simulink model "solar_collector"  (R2025b)
settings: Solver=ode15s  StartTime=0  StopTime=LP.duration  MaxStep=5  RelTol=1e-7  AbsTol=1e-7
values from neighbouring files (symbols this model uses):
  P = g.P    [simulate_collector.m]
undefined symbols (not defined in the file or in its folder): LP
settings Model: Creator=aevamac  LastModifiedBy=aevamac
settings DataIOCC: SaveFormat=Array  OutputOption=SpecifiedOutputTimes  OutputTimes=LP.out_times

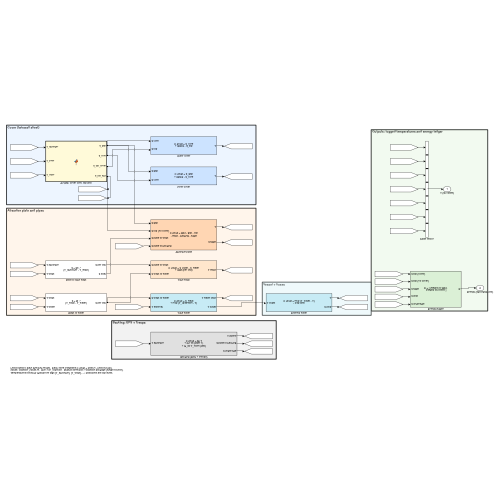
[thumbnail: Simulink's stored preview of the top-level diagram]
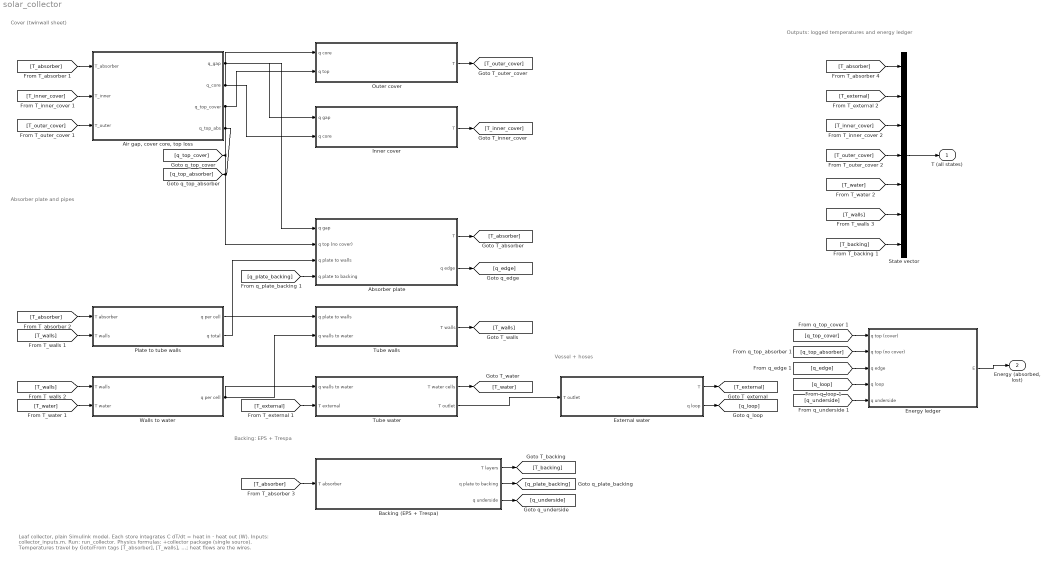
== system solar_collector ==
  note: Cover (twinwall sheet)
  note: Absorber plate and pipes
  note: Vessel + hoses
  note: Backing: EPS + Trespa
  note: Outputs: logged temperatures and energy ledger
  note: Leaf collector, plain Simulink model.  Each store integrates C dT/dt = heat in - heat out (W).
      | Inputs: collector_inputs.m.  Run: run_collector.  Physics formulas: +collector package (single source).
      | Temperatures travel by Goto/From tags [T_absorber], [T_walls], ...; heat flows are the wires.
  Absorber plate : Subsystem  Description=Aluminium plate + paint + tee fittings, one temperature. C dT/dt = (q_solar - q_tube) - q_gap - q_top(no cover) - sum q_plate->walls - q_plate->backing - edge loss
      mask Display:
      | disp(sprintf('C dT/dt = light - gap - top\n- walls - backing - edge'));
      | port_label('input', 1, 'q gap');
      | port_label('input', 2, 'q top (no cover)');
      | port_label('input', 3, 'q plate to walls');
      | port_label('input', 4, 'q plate to backing');
      | port_label('output', 1, 'T');
      | port_label('output', 2, 'q edge');
  "Air gap, cover core, top loss" : MATLAB Function  Description=Nonlinear surface heat flows from collector.surface_heat_flows: gap convection (Hollands-type correlation) + radiation, twinwall core conduction, and top loss by convection + radiation.  TreatAsAtomicUnit=on
  Backing (EPS + Trespa) : Subsystem  Description=EPS then the cart Trespa plate, each split into layers that store heat. Conduction plate -> layer 1 -> ... -> last layer -> underside air. Heat into the layers = Ab*Tb + G1*Ta (first) + G_air*T_room (last).
      mask Display:
      | disp(sprintf('C dT/dt = Ab T\n+ G1 Ta (layer 1)\n+ G_air T_room (last)'));
      | port_label('input', 1, 'T absorber');
      | port_label('output', 1, 'T layers');
      | port_label('output', 2, 'q plate to backing');
      | port_label('output', 3, 'q underside');
  Energy ledger : Subsystem  Description=Energy absorbed (light) and lost (top, edges, loop, underside), integrated so that absorbed - lost - stored can be checked (should be ~0).
      mask Display:
      | disp(sprintf('E = [ integral of light,\n integral of losses ]'));
      | port_label('input', 1, 'q top (cover)');
      | port_label('input', 2, 'q top (no cover)');
      | port_label('input', 3, 'q edge');
      | port_label('input', 4, 'q loop');
      | port_label('input', 5, 'q underside');
      | port_label('output', 1, 'E');
  External water : Subsystem  Description=Vessel and hoses, one mixed temperature. C dT/dt = mcp (T_outlet - Te) - loop_ua (Te - T_room)
      mask Display:
      | disp(sprintf('C dT/dt = mcp (T_outlet - T)\n- loop loss'));
      | port_label('input', 1, 'T outlet');
      | port_label('output', 1, 'T');
      | port_label('output', 2, 'q loop');
  Inner cover : Subsystem  Description=Inner cover sheet: C dT/dt = q_gap + q_cover/2 - q_core
      mask Display:
      | disp(sprintf('C dT/dt = q_gap\n+ light/2 - q_core'));
      | port_label('input', 1, 'q gap');
      | port_label('input', 2, 'q core');
      | port_label('output', 1, 'T');
  Outer cover : Subsystem  Description=Outer cover sheet: C dT/dt = q_core + q_cover/2 - q_top
      mask Display:
      | disp(sprintf('C dT/dt = q_core\n+ light/2 - q_top'));
      | port_label('input', 1, 'q core');
      | port_label('input', 2, 'q top');
      | port_label('output', 1, 'T');
  Plate to tube walls : Subsystem  Description=q = ga .* (T_absorber - T_walls), per cell; also the total leaving the plate
      mask Display:
      | disp(sprintf('q = ga .*\n(T_absorber - T_walls)'));
      | port_label('input', 1, 'T absorber');
      | port_label('input', 2, 'T walls');
      | port_label('output', 1, 'q per cell');
      | port_label('output', 2, 'q total');
  State vector : Concatenate  NumInputs=7
  Tube walls : Subsystem  Description=One LDPE wall cell per water cell. C dT/dt = ga(Ta - Tw) - gf(Tw - Tq) + light landing on the pipes (footprint share)
      mask Display:
      | disp(sprintf('C dT/dt = q_plate - q_water\n+ light (per cell)'));
      | port_label('input', 1, 'q plate to walls');
      | port_label('input', 2, 'q walls to water');
      | port_label('output', 1, 'T walls');
  Tube water : Subsystem  Description=Water cells in flow order (supply tiers, then the mirrored return). C dT/dt = gf(Tw - Tq) + mcp (T_upstream - Tq); the first cell is fed from the external water.
      mask Display:
      | disp(sprintf('C dT/dt = q_walls\n+ mcp (T_upstream - T)'));
      | port_label('input', 1, 'q walls to water');
      | port_label('input', 2, 'T external');
      | port_label('output', 1, 'T water cells');
      | port_label('output', 2, 'T outlet');
  Walls to water : Subsystem  Description=q = gf .* (T_walls - T_water), per cell
      mask Display:
      | disp(sprintf('q = gf .*\n(T_walls - T_water)'));
      | port_label('input', 1, 'T walls');
      | port_label('input', 2, 'T water');
      | port_label('output', 1, 'q per cell');
  T (all states) : Outport
  "Energy (absorbed, lost)" : Outport  Port=2
  wires:
  [T_absorber] -> "Air gap, cover core, top loss"/1(T_absorber)
  [T_inner_cover] -> "Air gap, cover core, top loss"/2(T_inner)
  [T_outer_cover] -> "Air gap, cover core, top loss"/3(T_outer)
  "Air gap, cover core, top loss"/1(q_gap) -> Inner cover/1(q gap), Absorber plate/1(q gap)
  "Air gap, cover core, top loss"/2(q_core) -> Inner cover/2(q core), Outer cover/1(q core)
  "Air gap, cover core, top loss"/3(q_top_cover) -> Outer cover/2(q top), [q_top_cover]
  Outer cover/1(T) -> [T_outer_cover]
  Inner cover/1(T) -> [T_inner_cover]
  "Air gap, cover core, top loss"/4(q_top_abs) -> [q_top_absorber], Absorber plate/2(q top (no cover))
  Absorber plate/1(T) -> [T_absorber]
  Absorber plate/2(q edge) -> [q_edge]
  [q_plate_backing] -> Absorber plate/4(q plate to backing)
  [T_absorber] -> Plate to tube walls/1(T absorber)
  [T_walls] -> Plate to tube walls/2(T walls)
  Plate to tube walls/1(q per cell) -> Tube walls/1(q plate to walls)
  Plate to tube walls/2(q total) -> Absorber plate/3(q plate to walls)
  Tube walls/1(T walls) -> [T_walls]
  [T_walls] -> Walls to water/1(T walls)
  [T_water] -> Walls to water/2(T water)
  Walls to water/1(q per cell) -> Tube walls/2(q walls to water), Tube water/1(q walls to water)
  [T_external] -> Tube water/2(T external)
  Tube water/1(T water cells) -> [T_water]
  Tube water/2(T outlet) -> External water/1(T outlet)
  External water/1(T) -> [T_external]
  External water/2(q loop) -> [q_loop]
  [T_absorber] -> Backing (EPS + Trespa)/1(T absorber)
  Backing (EPS + Trespa)/1(T layers) -> [T_backing]
  Backing (EPS + Trespa)/2(q plate to backing) -> [q_plate_backing]
  Backing (EPS + Trespa)/3(q underside) -> [q_underside]
  [q_top_cover] -> Energy ledger/1(q top (cover))
  [q_top_absorber] -> Energy ledger/2(q top (no cover))
  [q_edge] -> Energy ledger/3(q edge)
  [q_loop] -> Energy ledger/4(q loop)
  [q_underside] -> Energy ledger/5(q underside)
  Energy ledger/1(E) -> "Energy (absorbed, lost)"/1
  [T_absorber] -> State vector/1
  [T_external] -> State vector/2
  [T_inner_cover] -> State vector/3
  [T_outer_cover] -> State vector/4
  [T_water] -> State vector/5
  [T_walls] -> State vector/6
  [T_backing] -> State vector/7
  State vector/1 -> T (all states)/1

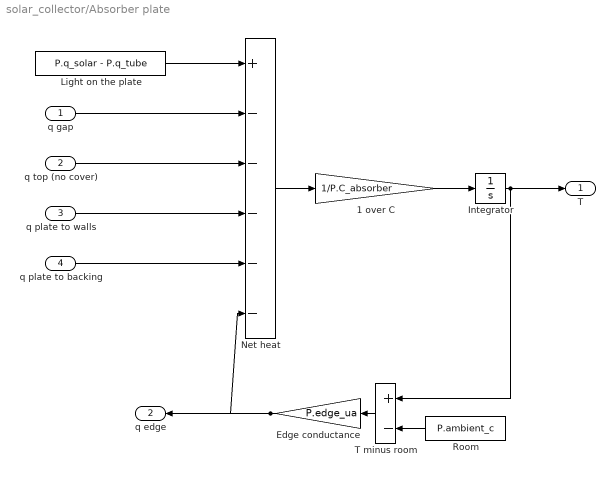
== system solar_collector/Absorber plate ==
  q gap : Inport
  q top (no cover) : Inport  Port=2
  q plate to walls : Inport  Port=3
  q plate to backing : Inport  Port=4
  1 over C : Gain  Gain=1/P.C_absorber
  Edge conductance : Gain  Gain=P.edge_ua
  Integrator : Integrator  InitialCondition=P.T0
  Light on the plate : Constant  Value=P.q_solar - P.q_tube
  Net heat : Sum  Inputs=+-----
  Room : Constant  Value=P.ambient_c
  T minus room : Sum  Inputs=+-
  T : Outport
  q edge : Outport  Port=2
  wires:
  Light on the plate/1 -> Net heat/1
  q gap/1 -> Net heat/2
  q top (no cover)/1 -> Net heat/3
  q plate to walls/1 -> Net heat/4
  q plate to backing/1 -> Net heat/5
  Net heat/1 -> 1 over C/1
  1 over C/1 -> Integrator/1
  Integrator/1 -> T/1, T minus room/1
  Room/1 -> T minus room/2
  T minus room/1 -> Edge conductance/1
  Edge conductance/1 -> Net heat/6, q edge/1

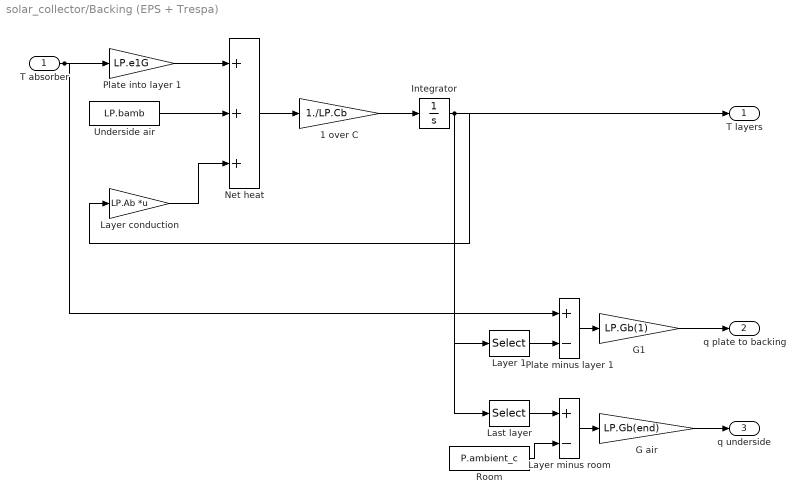
== system solar_collector/Backing (EPS + Trespa) ==
  T absorber : Inport
  1 over C : Gain  Gain=1./LP.Cb
  G air : Gain  Gain=LP.Gb(end)
  G1 : Gain  Gain=LP.Gb(1)
  Integrator : Integrator  InitialCondition=P.T0*ones(LP.nb,1)
  Last layer : Selector  InputPortWidth=LP.nb  IndexOptions=Index vector (dialog)  Indices=LP.nb  OutputSizes=1
  Layer 1 : Selector  InputPortWidth=LP.nb  IndexOptions=Index vector (dialog)  Indices=1  OutputSizes=1
  Layer conduction : Gain  Gain=LP.Ab  Multiplication=Matrix(K*u)
  Layer minus room : Sum  Inputs=+-
  Net heat : Sum  Inputs=+++
  Plate into layer 1 : Gain  Gain=LP.e1G
  Plate minus layer 1 : Sum  Inputs=+-
  Room : Constant  Value=P.ambient_c
  Underside air : Constant  Value=LP.bamb
  T layers : Outport
  q plate to backing : Outport  Port=2
  q underside : Outport  Port=3
  wires:
  Net heat/1 -> 1 over C/1
  1 over C/1 -> Integrator/1
  T absorber/1 -> Plate into layer 1/1, Plate minus layer 1/1
  Plate into layer 1/1 -> Net heat/1
  Underside air/1 -> Net heat/2
  Layer conduction/1 -> Net heat/3
  Integrator/1 -> T layers/1, Layer conduction/1, Layer 1/1, Last layer/1
  Layer 1/1 -> Plate minus layer 1/2
  Plate minus layer 1/1 -> G1/1
  G1/1 -> q plate to backing/1
  Last layer/1 -> Layer minus room/1
  Room/1 -> Layer minus room/2
  Layer minus room/1 -> G air/1
  G air/1 -> q underside/1

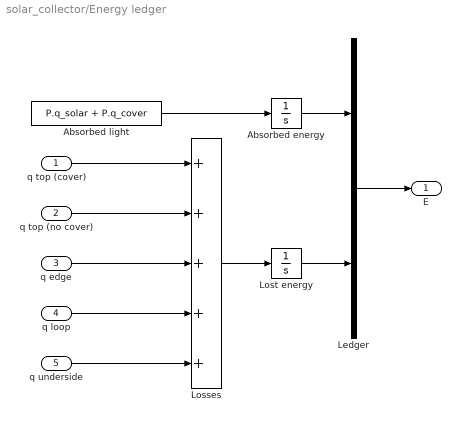
== system solar_collector/Energy ledger ==
  q top (cover) : Inport
  q top (no cover) : Inport  Port=2
  q edge : Inport  Port=3
  q loop : Inport  Port=4
  q underside : Inport  Port=5
  Absorbed energy : Integrator
  Absorbed light : Constant  Value=P.q_solar + P.q_cover
  Ledger : Mux  Inputs=2
  Losses : Sum  Inputs=+++++
  Lost energy : Integrator
  E : Outport
  wires:
  q top (cover)/1 -> Losses/1
  q top (no cover)/1 -> Losses/2
  q edge/1 -> Losses/3
  q loop/1 -> Losses/4
  q underside/1 -> Losses/5
  Absorbed light/1 -> Absorbed energy/1
  Losses/1 -> Lost energy/1
  Absorbed energy/1 -> Ledger/1
  Lost energy/1 -> Ledger/2
  Ledger/1 -> E/1

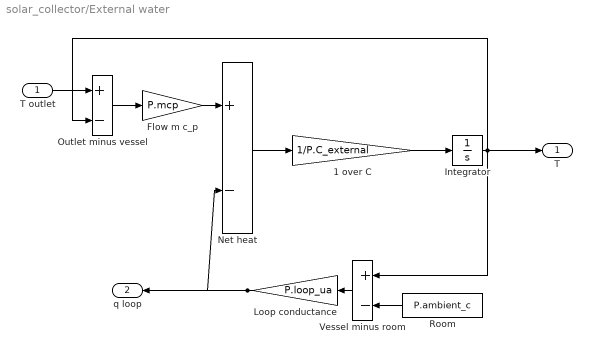
== system solar_collector/External water ==
  T outlet : Inport
  1 over C : Gain  Gain=1/P.C_external
  Flow m c_p : Gain  Gain=P.mcp
  Integrator : Integrator  InitialCondition=P.T0
  Loop conductance : Gain  Gain=P.loop_ua
  Net heat : Sum  Inputs=+-
  Outlet minus vessel : Sum  Inputs=+-
  Room : Constant  Value=P.ambient_c
  Vessel minus room : Sum  Inputs=+-
  T : Outport
  q loop : Outport  Port=2
  wires:
  Net heat/1 -> 1 over C/1
  1 over C/1 -> Integrator/1
  T outlet/1 -> Outlet minus vessel/1
  Outlet minus vessel/1 -> Flow m c_p/1
  Flow m c_p/1 -> Net heat/1
  Integrator/1 -> T/1, Outlet minus vessel/2, Vessel minus room/1
  Room/1 -> Vessel minus room/2
  Vessel minus room/1 -> Loop conductance/1
  Loop conductance/1 -> Net heat/2, q loop/1

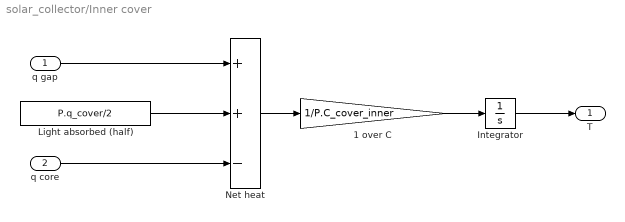
== system solar_collector/Inner cover ==
  q gap : Inport
  q core : Inport  Port=2
  1 over C : Gain  Gain=1/P.C_cover_inner
  Integrator : Integrator  InitialCondition=P.T0
  Light absorbed (half) : Constant  Value=P.q_cover/2
  Net heat : Sum  Inputs=++-
  T : Outport
  wires:
  q gap/1 -> Net heat/1
  Light absorbed (half)/1 -> Net heat/2
  q core/1 -> Net heat/3
  Net heat/1 -> 1 over C/1
  1 over C/1 -> Integrator/1
  Integrator/1 -> T/1

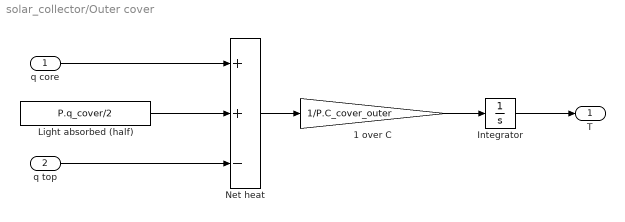
== system solar_collector/Outer cover ==
  q core : Inport
  q top : Inport  Port=2
  1 over C : Gain  Gain=1/P.C_cover_outer
  Integrator : Integrator  InitialCondition=P.T0
  Light absorbed (half) : Constant  Value=P.q_cover/2
  Net heat : Sum  Inputs=++-
  T : Outport
  wires:
  q core/1 -> Net heat/1
  Light absorbed (half)/1 -> Net heat/2
  q top/1 -> Net heat/3
  Net heat/1 -> 1 over C/1
  1 over C/1 -> Integrator/1
  Integrator/1 -> T/1

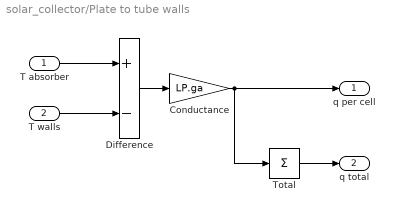
== system solar_collector/Plate to tube walls ==
  T absorber : Inport
  T walls : Inport  Port=2
  Conductance : Gain  Gain=LP.ga
  Difference : Sum  Inputs=+-
  Total : Sum  Inputs=+
  q per cell : Outport
  q total : Outport  Port=2
  wires:
  T absorber/1 -> Difference/1
  T walls/1 -> Difference/2
  Difference/1 -> Conductance/1
  Conductance/1 -> q per cell/1, Total/1
  Total/1 -> q total/1

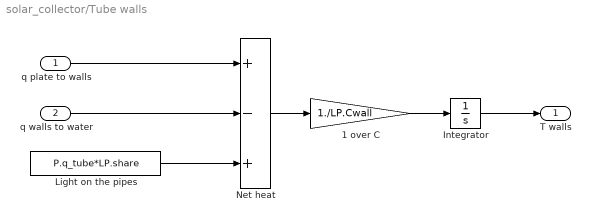
== system solar_collector/Tube walls ==
  q plate to walls : Inport
  q walls to water : Inport  Port=2
  1 over C : Gain  Gain=1./LP.Cwall
  Integrator : Integrator  InitialCondition=P.T0*ones(LP.nw,1)
  Light on the pipes : Constant  Value=P.q_tube*LP.share
  Net heat : Sum  Inputs=+-+
  T walls : Outport
  wires:
  q plate to walls/1 -> Net heat/1
  q walls to water/1 -> Net heat/2
  Light on the pipes/1 -> Net heat/3
  Net heat/1 -> 1 over C/1
  1 over C/1 -> Integrator/1
  Integrator/1 -> T walls/1

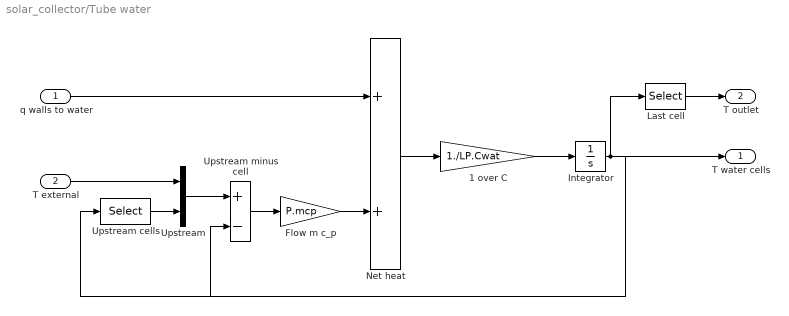
== system solar_collector/Tube water ==
  q walls to water : Inport
  T external : Inport  Port=2
  1 over C : Gain  Gain=1./LP.Cwat
  Flow m c_p : Gain  Gain=P.mcp
  Integrator : Integrator  InitialCondition=P.T0*ones(LP.nw,1)
  Last cell : Selector  InputPortWidth=LP.nw  IndexOptions=Index vector (dialog)  Indices=LP.nw  OutputSizes=1
  Net heat : Sum
  Upstream : Concatenate
  Upstream cells : Selector  InputPortWidth=LP.nw  IndexOptions=Index vector (dialog)  Indices=1:LP.nw-1  OutputSizes=1
  Upstream minus cell : Sum  Inputs=+-
  T water cells : Outport
  T outlet : Outport  Port=2
  wires:
  Net heat/1 -> 1 over C/1
  1 over C/1 -> Integrator/1
  q walls to water/1 -> Net heat/1
  T external/1 -> Upstream/1
  Upstream cells/1 -> Upstream/2
  Upstream/1 -> Upstream minus cell/1
  Upstream minus cell/1 -> Flow m c_p/1
  Flow m c_p/1 -> Net heat/2
  Integrator/1 -> T water cells/1, Last cell/1, Upstream cells/1, Upstream minus cell/2
  Last cell/1 -> T outlet/1

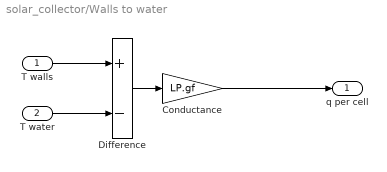
== system solar_collector/Walls to water ==
  T walls : Inport
  T water : Inport  Port=2
  Conductance : Gain  Gain=LP.gf
  Difference : Sum  Inputs=+-
  q per cell : Outport
  wires:
  T walls/1 -> Difference/1
  T water/1 -> Difference/2
  Difference/1 -> Conductance/1
  Conductance/1 -> q per cell/1

== matlab function solar_collector/Air gap, cover core, top loss ==
  data: T_absorber input double size=1; q_gap output double size=1; T_inner input double size=1; T_outer input double size=1; q_core output double size=1; q_top_cover output double size=1; q_top_abs output double size=1; P parameter
function [q_gap, q_core, q_top_cover, q_top_abs] = f(T_absorber, T_inner, T_outer, P)
% Heat flows (W) above the absorber; formulas in +collector/surface_heat_flows.m
[q_gap, q_core, q_top_cover, q_top_abs] = collector.surface_heat_flows(T_absorber, T_inner, T_outer, P);
